simulink model "robc_mmc_simult"  (R2024b)
settings: Solver=FixedStepAuto  StartTime=0.0  StopTime=TSim  FixedStep=Ts  RelTol=1e-3
InitFcn:
  | load('fbg_controller_parameters.mat')
  | load('fb_controller_parameters.mat')
  | load('ff_controller_parameters.mat')
  | load('ss_model_parameters.mat')
  | load('operating_point_parameters.mat')
  | integralFlag = 1;
values from neighbouring files (symbols this model uses):
  Id_ref = 0    [main_simk_ccc.m]    (also in main_simk_occ.m = 1; main_simk_s.m = 1; operating_point_c_parameters.mat; operating_point_parameters.mat = 1)
  Iq_ref = 0    [main_simk_ccc.m]    (also in main_simk_occ.m; main_simk_s.m; operating_point_c_parameters.mat; operating_point_parameters.mat)
  Ts = 5e-05    [LoadParameters_SFC2K.mat]    (also in fb_c_controller_parameters.mat; fb_controller_parameters.mat; fbg_c_controller_parameters.mat; fbg_controller_parameters.mat)
  ulim = 1.2    [main_simk_ccc.m]    (also in main_simk_occ.m; main_simk_s.m; operating_point_c_parameters.mat; operating_point_parameters.mat)
  Vd_ = 0    [main_simk_ccc.m]    (also in main_simk_occ.m; main_simk_s.m; operating_point_c_parameters.mat; operating_point_parameters.mat)
  Vq_ = 0    [main_simk_ccc.m]    (also in main_simk_occ.m; main_simk_s.m; operating_point_c_parameters.mat; operating_point_parameters.mat)
undefined symbols (not defined in the file or in its folder): DiscIntNeverNeededParam
settings Model: Creator=rmrane  LastModifiedBy=vreyesdreke
settings OptimizationCC: DefaultParameterBehavior=Inlined  EnhancedBackFolding=on  PassReuseOutputArgsAs=Individual arguments  ZeroExternalMemoryAtStartup=off  ZeroInternalMemoryAtStartup=off  OptimizeBlockOrder=speed  DifferentSizesBufferReuse=on  OptimizationCustomize=off  EfficientTunableParamExpr=on
settings DebuggingCC: ParameterTunabilityLossMsg=error
settings SFSimCC: MATLABDynamicMemAlloc=off
settings RTWCC: Description=Embedded Coder  SystemTargetFile=ert.tlc  TemplateMakefile=ert_default_tmf
settings CodeAppCC: GenerateComments=off  IgnoreCustomStorageClasses=off  OperatorAnnotations=on  SimulinkDataObjDesc=on  SFDataObjDesc=on  CustomSymbolStrType=$N$R$M  SimulinkBlockComments=off  InternalIdentifier=Classic
settings ERTTargetCC: GenerateSampleERTMain=on  SupportAbsoluteTime=off  SupportNonFinite=off  SupportComplex=off  ERTCustomFileTemplate=example_file_process.tlc  ConvertIfToSwitch=off  SuppressUnreachableDefaultCases=off  EnableSignedLeftShifts=off  EnableSignedRightShifts=off  DynamicArrayContainerType=coder::array

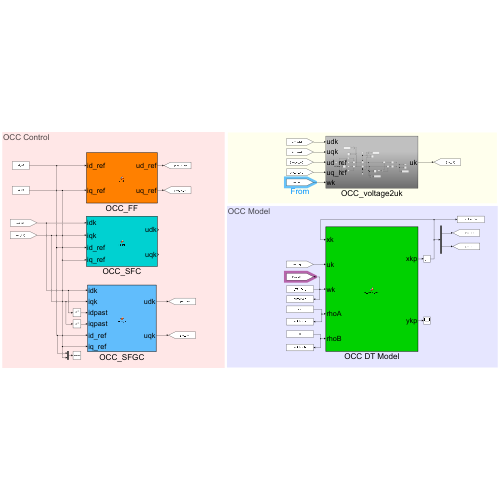
[thumbnail: Simulink's stored preview of the top-level diagram]
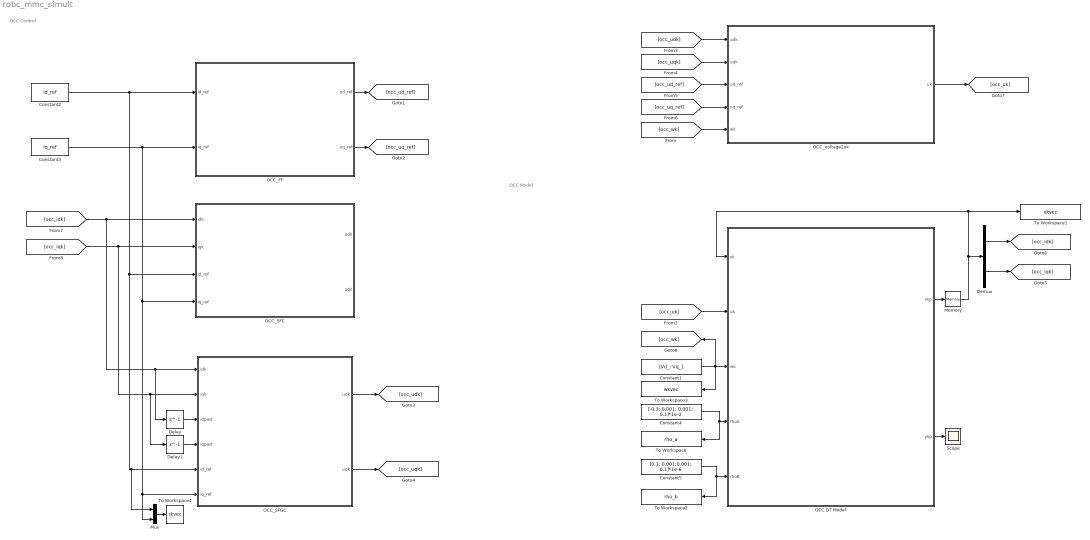
== system robc_mmc_simult ==
  note: OCC Model
  note: OCC Control
  Constant1 : Constant  Value=[Vd_; Vq_]  SampleTime=Ts
  Constant2 : Constant  Value=Id_ref  SampleTime=Ts
  Constant3 : Constant  Value=Iq_ref  SampleTime=Ts
  Constant4 : Constant  Value=[-0.3; 0.001; 0.001; 0.1]*1e-2  SampleTime=Ts
  Constant5 : Constant  Value=[0.1; 0.001;0.001; 0.1]*1e-6  SampleTime=Ts
  Delay : Delay  DelayLength=1  InputProcessing=Columns as channels (frame based)  SampleTime=Ts
  Delay1 : Delay  DelayLength=1  InputProcessing=Columns as channels (frame based)  SampleTime=Ts
  Demux : Demux  Outputs=2
  Memory : Memory  InheritSampleTime=on  LinearizeAsDelay=on
  Mux : Mux  Inputs=2
  OCC DT Model : MATLAB Function  TreatAsAtomicUnit=on
  OCC_FF : MATLAB Function  TreatAsAtomicUnit=on
  OCC_SFC : MATLAB Function  TreatAsAtomicUnit=on
  OCC_SFGC : MATLAB Function  TreatAsAtomicUnit=on
  OCC_voltage2uk : Subsystem
  Scope : Scope
  To Workspace : ToWorkspace  VariableName=rho_a  SampleTime=Ts
      settings: Save2DSignal=2-D array (concatenate along first dimension)
  To Workspace1 : ToWorkspace  VariableName=xkvec  SampleTime=Ts
      settings: Save2DSignal=2-D array (concatenate along first dimension)
  To Workspace2 : ToWorkspace  VariableName=rho_b  SampleTime=Ts
      settings: Save2DSignal=2-D array (concatenate along first dimension)
  To Workspace3 : ToWorkspace  VariableName=wkvec  SampleTime=Ts
      settings: Save2DSignal=2-D array (concatenate along first dimension)
  To Workspace4 : ToWorkspace  VariableName=rkvec  SampleTime=Ts
      settings: Save2DSignal=2-D array (concatenate along first dimension)
  wires:
  Constant1/1 -> [occ_wk], To Workspace3/1, OCC DT Model/3(wk)
  OCC DT Model/1(xkp) -> Memory/1
  OCC_FF/1(ud_ref) -> [occ_ud_ref]
  OCC_FF/2(uq_ref) -> [occ_uq_ref]
  Constant2/1 -> OCC_FF/1(id_ref), Mux/1, OCC_SFGC/5(id_ref), OCC_SFC/3(id_ref)
  Constant3/1 -> OCC_FF/2(iq_ref), Mux/2, OCC_SFGC/6(iq_ref), OCC_SFC/4(iq_ref)
  Memory/1 -> Demux/1, To Workspace1/1, OCC DT Model/1(xk)
  Demux/2 -> [occ_iqk]
  Demux/1 -> [occ_idk]
  OCC_voltage2uk/1(uk) -> [occ_uk]
  [occ_uk] -> OCC DT Model/2(uk)
  [occ_udk] -> OCC_voltage2uk/1(udk)
  [occ_uqk] -> OCC_voltage2uk/2(uqk)
  [occ_ud_ref] -> OCC_voltage2uk/3(ud_ref)
  [occ_uq_ref] -> OCC_voltage2uk/4(uq_ref)
  [occ_idk] -> Delay/1, OCC_SFGC/1(idk), OCC_SFC/1(idk)
  [occ_iqk] -> Delay1/1, OCC_SFGC/2(iqk), OCC_SFC/2(iqk)
  Constant4/1 -> To Workspace/1, OCC DT Model/4(rhoA)
  Constant5/1 -> To Workspace2/1, OCC DT Model/5(rhoB)
  OCC DT Model/2(ykp) -> Scope/1
  Delay/1 -> OCC_SFGC/3(idpast)
  Delay1/1 -> OCC_SFGC/4(iqpast)
  OCC_SFGC/2(uqk) -> [occ_uqk]
  OCC_SFGC/1(udk) -> [occ_udk]
  Mux/1 -> To Workspace4/1
  [occ_wk] -> OCC_voltage2uk/5(wk)

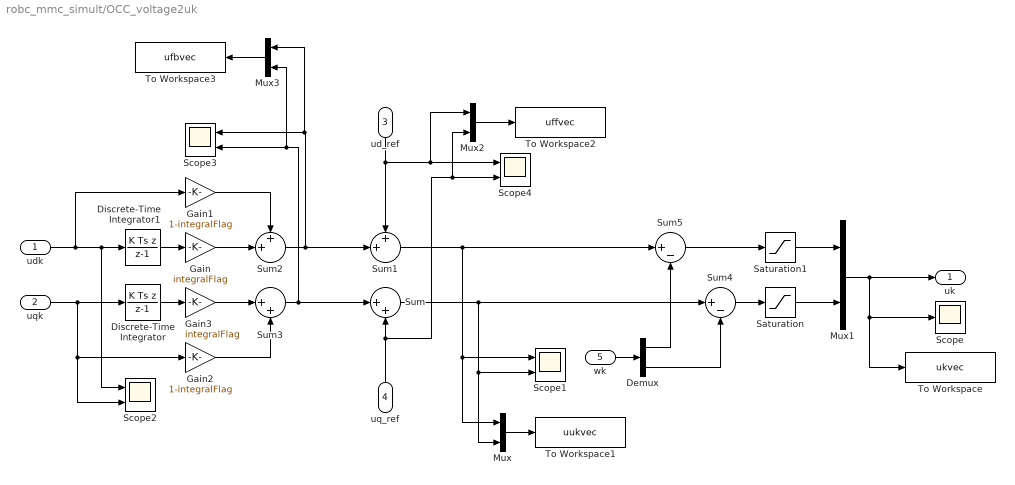
== system robc_mmc_simult/OCC_voltage2uk ==
  udk : Inport
  uqk : Inport  Port=2
  ud_ref : Inport  Port=3
  uq_ref : Inport  Port=4
  wk : Inport  Port=5
  Demux : Demux  Outputs=2
  Discrete-Time Integrator : DiscreteIntegrator  IntegratorMethod=Integration: Backward Euler  gainval=1.0/Ts  SampleTime=Ts  ICPrevOutput=DiscIntNeverNeededParam  ICPrevScaledInput=DiscIntNeverNeededParam
  Discrete-Time Integrator1 : DiscreteIntegrator  IntegratorMethod=Integration: Backward Euler  gainval=1.0/Ts  SampleTime=Ts  ICPrevOutput=DiscIntNeverNeededParam  ICPrevScaledInput=DiscIntNeverNeededParam
  Gain : Gain  Gain=integralFlag
  Gain1 : Gain  Gain=1-integralFlag
  Gain2 : Gain  Gain=1-integralFlag
  Gain3 : Gain  Gain=integralFlag
  Mux{,1..3} (4 alike) : Mux  Inputs=2
  Saturation : Saturate  UpperLimit=ulim  LowerLimit=-ulim
  Saturation1 : Saturate  UpperLimit=ulim  LowerLimit=-ulim
  Scope : Scope
  Scope{1..4} (4 alike) : Scope  NumInputPorts=2
  Sum : Sum  Inputs=|++
  Sum1 : Sum  Inputs=++|
  Sum2 : Sum  Inputs=++|
  Sum3 : Sum  Inputs=|++
  Sum4 : Sum  Inputs=|+-
  Sum5 : Sum  Inputs=|+-
  To Workspace : ToWorkspace  VariableName=ukvec  SampleTime=Ts
      settings: Save2DSignal=2-D array (concatenate along first dimension)
  To Workspace1 : ToWorkspace  VariableName=uukvec  SampleTime=Ts
      settings: Save2DSignal=2-D array (concatenate along first dimension)
  To Workspace2 : ToWorkspace  VariableName=uffvec  SampleTime=Ts
      settings: Save2DSignal=2-D array (concatenate along first dimension)
  To Workspace3 : ToWorkspace  VariableName=ufbvec  SampleTime=Ts
      settings: Save2DSignal=2-D array (concatenate along first dimension)
  uk : Outport
  wires:
  Sum2/1 -> Mux3/1, Scope3/1, Sum1/2
  Gain2/1 -> Sum3/2
  uq_ref/1 -> Mux2/2, Scope4/2, Sum/2
  ud_ref/1 -> Mux2/1, Scope4/1, Sum1/1
  udk/1 -> Scope2/1, Discrete-Time Integrator1/1, Gain1/1
  Discrete-Time Integrator1/1 -> Gain/1
  Sum/1 -> Sum4/1, Mux/2, Scope1/2
  Sum3/1 -> Mux3/2, Scope3/2, Sum/1
  Saturation/1 -> Mux1/2
  Mux1/1 -> To Workspace/1, Scope/1, uk/1
  Gain/1 -> Sum2/2
  Gain3/1 -> Sum3/1
  Saturation1/1 -> Mux1/1
  Sum1/1 -> Sum5/1, Mux/1, Scope1/1
  Discrete-Time Integrator/1 -> Gain3/1
  uqk/1 -> Scope2/2, Gain2/1, Discrete-Time Integrator/1
  Gain1/1 -> Sum2/1
  Mux/1 -> To Workspace1/1
  Mux2/1 -> To Workspace2/1
  Mux3/1 -> To Workspace3/1
  wk/1 -> Demux/1
  Demux/2 -> Sum4/2
  Demux/1 -> Sum5/2
  Sum5/1 -> Saturation1/1
  Sum4/1 -> Saturation/1

== matlab function robc_mmc_simult/OCC DT Model ==
  settings: updateMethod=DISCRETE  sampleTime=Ts
  data: xk input size=2; xkp output size=2; uk input size=2; ykp output size=2; wk input size=2; rhoA input size=4; rhoB input size=4
function [xkp,ykp] = dt_model_occ(xk, uk, wk, rhoA, rhoB)
% dt_model_occ(xk, uk, wk) discrete-time model of the MMC OCC dynamics.
    m_ss = coder.load('ss_model_parameters.mat','-mat','-regexp',...
        'A','B','C','D','E');
    dA = [rhoA(1), rhoA(2); rhoA(3), rhoA(4)];
    dB = [rhoB(1), rhoB(2); rhoB(3), rhoB(4)];
    xkp = (m_ss.A+dA)*xk+(m_ss.B+dB)*uk+m_ss.E*wk;
    ykp = m_ss.C*xk;
end

== matlab function robc_mmc_simult/OCC_SFC ==
  settings: updateMethod=DISCRETE  sampleTime=Ts
  data: idk input size=1; udk output size=1; iqk input size=1; uqk output size=1; id_ref input; iq_ref input
function [udk,uqk] = oc_sfc(idk, iqk,id_ref,iq_ref)
    % oc_sfc(idk, iqk,id_ref,iq_ref) feedforward controller gain.
    m_ss = coder.load('fb_controller_parameters.mat','-mat','-regexp','Kfb');
    uk = m_ss.Kfb*([idk, iqk]'-[id_ref,iq_ref]');
    udk = uk(1);
    uqk = uk(2);
end

== matlab function robc_mmc_simult/OCC_FF ==
  settings: updateMethod=DISCRETE  sampleTime=Ts
  data: id_ref input size=1; ud_ref output size=1; iq_ref input size=1; uq_ref output size=1
function [ud_ref,uq_ref] = oc_ffc(id_ref,iq_ref)
    % oc_ffc(id_ref,iq_ref) feedforward controller gain.
    m_ss = coder.load('ff_controller_parameters.mat','-mat','-regexp','Kff');
    uss = m_ss.Kff*[id_ref,iq_ref]';
    ud_ref = uss(1);
    uq_ref = uss(2);
end

== matlab function robc_mmc_simult/OCC_SFGC ==
  settings: updateMethod=DISCRETE  sampleTime=Ts
  data: idk input size=1; udk output size=1; iqk input size=1; idpast input size=1; iqpast input size=1; uqk output size=1; id_ref input; iq_ref input
function [udk,uqk] = oc_sfgc(idk, iqk,idpast, iqpast,id_ref,iq_ref)
    % oc_sfc(idk, iqk,id_ref,iq_ref) feedforward controller gain.
    m_ss = coder.load('fbg_controller_parameters.mat','-mat','-regexp','Kfbg');
    ekvec = [(idk-idpast), (iqk-iqpast),idk,iqk]'-[0,0,id_ref,iq_ref]';
    uk = m_ss.Kfbg*ekvec;
    udk = uk(1);
    uqk = uk(2);
end
